simulink subsystem "force_to_pwm"  (R2026a)
settings: Solver=VariableStepAuto
undefined symbols (not defined in the file): P, S, T
PreSaveFcn:
  | defaultToFileBlockNames(bdroot);
settings Model: Creator=koryh  LastModifiedBy=kjhaydon

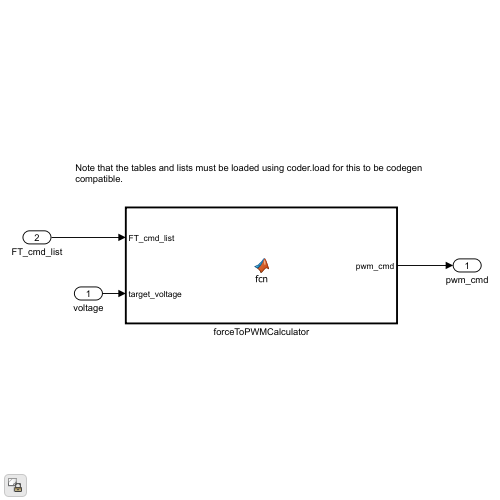
[thumbnail: Simulink's stored preview of the top-level diagram]
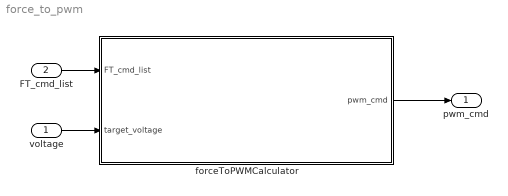
== system force_to_pwm ==
  voltage : Inport
  FT_cmd_list : Inport  Port=2  PortDimensions=[8,1]  SampleTime=S.dt_control
  forceToPWMCalculator : MATLAB Function  TreatAsAtomicUnit=on
  pwm_cmd : Outport
  wires:
  FT_cmd_list/1 -> forceToPWMCalculator/1(FT_cmd_list)
  forceToPWMCalculator/1(pwm_cmd) -> pwm_cmd/1
  voltage/1 -> forceToPWMCalculator/2(target_voltage)

== matlab function force_to_pwm/forceToPWMCalculator ==
  data: FT_cmd_list input; target_voltage input; pwm_cmd output size=[8 1]; P parameter; T parameter
function pwm_cmd = fcn(FT_cmd_list, target_voltage, P, T)

cw_pwm = P.Constants.cw_pwm;
ccw_pwm = P.Constants.ccw_pwm;
cw_force = P.Constants.cw_force;
ccw_force = P.Constants.ccw_force;
voltage = P.Constants.voltage;
pwm_upper_limit = T.pwm_upper_limit;
pwm_lower_limit = T.pwm_lower_limit;

pwm_cmd = forceToPWMCalculator(FT_cmd_list, target_voltage, cw_pwm, ccw_pwm, cw_force, ccw_force, voltage, pwm_upper_limit, pwm_lower_limit);
pwm_cmd = pwm_cmd(:);
